simulink model "arduino_serial_comentado_2021_slx_8_entradas"  (R2023b)
settings: Solver=VariableStepAuto  StartTime=0.0  StopTime=Inf  RelTol=1e-3
libraries: instrumentseriallib x3
settings Model: Creator=Claudio  LastModifiedBy=fjmoy
settings DebuggingCC: UnconnectedInputMsg=warning  UnconnectedOutputMsg=warning  UnconnectedLineMsg=warning
settings ModelReferenceCC: EnableRefExpFcnMdlSchedulingChecks=on
settings RTWCC: DLArmComputeVersion=19.05

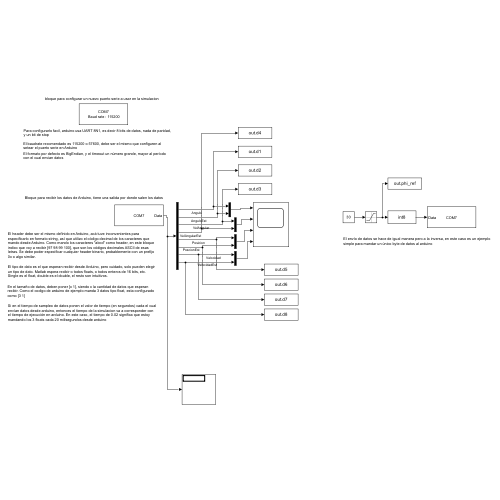
[thumbnail: Simulink's stored preview of the top-level diagram]
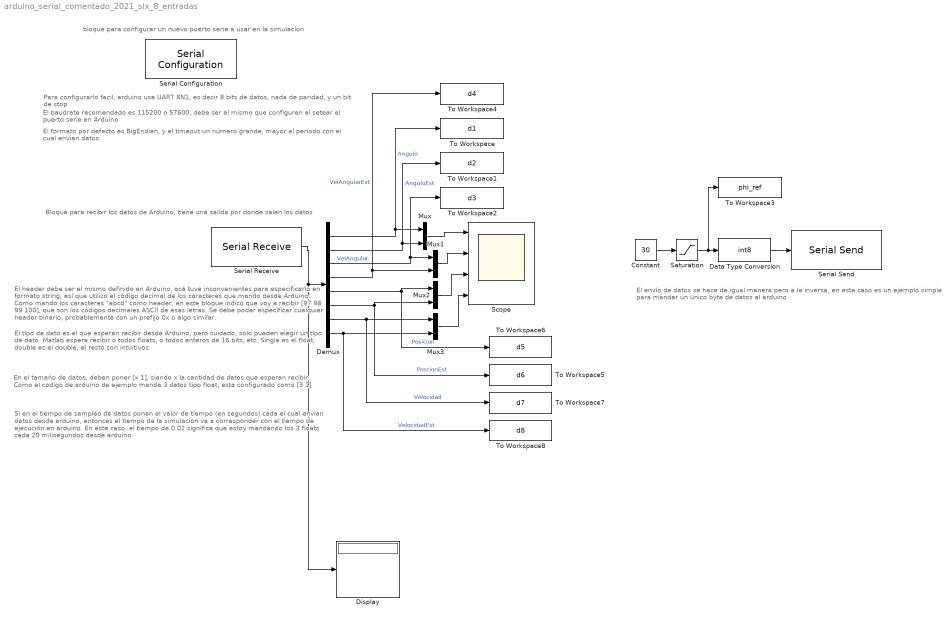
== system arduino_serial_comentado_2021_slx_8_entradas ==
  note: El envío de datos se hace de igual manera pero a la inversa, en este caso es un ejemplo simple para mandar un único byte de datos al arduino
  note: Si en el tiempo de sampleo de datos ponen el valor de tiempo (en segundos) cada el cual envían datos desde arduino, entonces el tiempo de la simulacion va a corresponder con el tiempo de ejecución en arduino. En este caso, el tiempo de 0.02 significa que estoy mandando los 3 floats cada 20 milisegundos desde arduino
  note: En el tamaño de datos, deben poner [x 1], siendo x la cantidad de datos que esperan recibir. Como el codigo de arduino de ejemplo manda 3 datos tipo float, esta configurado como [3 1]
  note: El tipo de dato es el que esperan recibir desde Arduino, pero cuidado, solo pueden elegir un tipo de dato. Matlab espera recibir o todos floats, o todos enteros de 16 bits, etc. Single es el float, double es el double, el resto son intuitivos.
  note: El header debe ser el mismo definido en Arduino, acá tuve inconvenientes para especificarlo en formato string, así que utilizo el código decimal de los caracteres que mando desde Arduino. Como mando los caracteres "abcd" como header, en este bloque indico que voy a recibir [97 98 99 100], que son los códigos decimales ASCII de esas letras. Se debe poder especificar cualquier header binario, probablemente con un prefijo 0x o algo similar.
  note: Bloque para recibir los datos de Arduino, tiene una salida por donde salen los datos
  note: El formato por defecto es BigEndian, y el timeout un número grande, mayor al período con el cual envian datos
  note: El baudrate recomendado es 115200 o 57600, debe ser el mismo que configuren al setear el puerto serie en Arduino
  note: Para configurarlo facil, arduino usa UART 8N1, es decir 8 bits de datos, nada de paridad, y un bit de stop
  note: bloque para configurar un nuevo puerto serie a usar en la simulacion
  Constant : Constant  Value=30
  Data Type Conversion : DataTypeConversion  OutDataTypeStr=int8  SaturateOnIntegerOverflow=off  RndMeth=Floor
  Demux : Demux  Outputs=8
  Display : Display
  Mux{,1..3} (4 alike) : Mux  Inputs=2
  Saturation : Saturate  UpperLimit=45  LowerLimit=-45
  Scope : Scope  NumInputPorts=4
  Serial Configuration : instrumentseriallib/Serial Configuration  Priority=-200000  PortSel=COM7  Port=COM7  ComPort=COM7  BaudRate=115200  DataBits=8  Parity=none  StopBits=1  ByteOrder=big-endian  FlowControl=none  Timeout=10  SimulateUsing=Interpreted execution  BlockInModel=on  aMode=1
  Serial Receive : instrumentseriallib/Serial Receive  Priority=1  PortSel=COM7  Port=COM7  ComPort=COM7  DataType=single  SaveDataType=uint8  ToggleHeader=on  Header="[ 97   98   99  100 ]"  ToggleTerminator=off  Terminator=<none>  CustomTerminator=[]  InputFormat=Column major  ToggleDataSize=on  DataSize=[8 1]  EnableBlockingMode=on  ActionDataUnavailable=Output last received value  ActionWhenDataUnavailable=Output last received value  CustomValue=0  SampleTime=0.02  SimulateUsing=Interpreted execution  BlockInModel=on  aMode=1
  Serial Send : instrumentseriallib/Serial Send  Priority=1  PortSel=COM7  Port=COM7  ComPort=COM7  Header=[]  Terminator=<none>  CustomTerminator=[]  EnableBlockingMode=on  SimulateUsing=Interpreted execution  BlockInModel=on  aMode=1
  To Workspace : ToWorkspace  VariableName=d1  SampleTime=-1
      settings: Save2DSignal=2-D array (concatenate along first dimension)
  To Workspace1 : ToWorkspace  VariableName=d2  SampleTime=-1
      settings: Save2DSignal=2-D array (concatenate along first dimension)
  To Workspace2 : ToWorkspace  VariableName=d3  SampleTime=-1
      settings: Save2DSignal=2-D array (concatenate along first dimension)
  To Workspace3 : ToWorkspace  VariableName=phi_ref  SampleTime=0.02
      settings: Save2DSignal=2-D array (concatenate along first dimension)
  To Workspace4 : ToWorkspace  VariableName=d4  SampleTime=-1
      settings: Save2DSignal=2-D array (concatenate along first dimension)
  To Workspace5 : ToWorkspace  VariableName=d6  SampleTime=-1
      settings: Save2DSignal=2-D array (concatenate along first dimension)
  To Workspace6 : ToWorkspace  VariableName=d5  SampleTime=-1
      settings: Save2DSignal=2-D array (concatenate along first dimension)
  To Workspace7 : ToWorkspace  VariableName=d7  SampleTime=-1
      settings: Save2DSignal=2-D array (concatenate along first dimension)
  To Workspace8 : ToWorkspace  VariableName=d8  SampleTime=-1
      settings: Save2DSignal=2-D array (concatenate along first dimension)
  wires:
  Demux/2 -> To Workspace1/1, Mux/2  "AnguloEst"
  Demux/1 -> Mux/1, To Workspace/1  "Angulo"
  Serial Receive/1 -> Display/1, Demux/1
  Demux/3 -> Mux1/1, To Workspace2/1  "VelAngular"
  Data Type Conversion/1 -> Serial Send/1
  Constant/1 -> Saturation/1
  Saturation/1 -> To Workspace3/1, Data Type Conversion/1
  Demux/4 -> To Workspace4/1, Mux1/2  "VelAngularEst"
  Mux/1 -> Scope/1
  Mux1/1 -> Scope/2
  Demux/5 -> To Workspace6/1, Mux2/1  "Posicion"
  Demux/6 -> To Workspace5/1, Mux2/2  "PoscionEst"
  Mux2/1 -> Scope/3
  Demux/7 -> To Workspace7/1, Mux3/1  "Velocidad"
  Demux/8 -> To Workspace8/1, Mux3/2  "VelocidadEst"
  Mux3/1 -> Scope/4
